simulink model "radia_ih"  (R2026a)
settings: Solver=FixedStepDiscrete  StopTime=1  FixedStep=0.10000000000000001
PreLoadFcn:
  | radia.simulink.makeIHMonitorBusObject();
InitFcn:
  | radia.simulink.updateIHGeometry(string(bdroot));
model workspace (MAT data in the model file):
  radia_ih_config.schema = 'radia.ih.simulink.native_sfunction.v1'
  radia_ih_config.backend = 'matlab-level2+radia-mex-handles'
  radia_ih_config.python_fallback = 0
  radia_ih_config.release_channel = "preview"
  radia_ih_config.operator_assembly = "diagnostic"
  radia_ih_config.diagnostic_only = 1
  radia_ih_config.eddy_solver = 'fem'
  radia_ih_config.thermal_solver = 'fem'
  radia_ih_config.n_eddy_unknown = 1
  radia_ih_config.n_heat = 1
  radia_ih_config.n_temperature = 1
  radia_ih_config.bh_mode = 'linear'
  radia_ih_config.eddy_matrix_real = 1
  radia_ih_config.eddy_matrix_imag = 0
  radia_ih_config.eddy_rhs_real = 1
  radia_ih_config.eddy_rhs_imag = 0
  radia_ih_config.heat_projection = 1
  radia_ih_config.heat_cell_weights = 1
  radia_ih_config.heat_to_temperature_projection = 1
  radia_ih_config.mass_row_ptr = [0; 1]
  radia_ih_config.mass_col = 0
  radia_ih_config.mass_value = 1
  radia_ih_config.stiffness_row_ptr = [0; 1]
  radia_ih_config.stiffness_col = 0
  radia_ih_config.stiffness_value = 0
  radia_ih_config.temperature_cell_weights = 1
  radia_ih_config.initial_temperature_K = 293.15
  radia_ih_config.sample_time_s = 0.1
  radia_ih_config.thermal_tolerance = 1e-12
  radia_ih_config.thermal_max_iterations = 100
  radia_ih_config.rotation_mode = 'periodic-uniform'
  radia_ih_config.angle_origin_rad = 0
  radia_ih_config.temperature_coordinate_system = "workpiece"
  radia_ih_config.rotation_transport = "conservative-periodic"
  radia_ih_config.dt_order = "eddy;transport(theta_prev,theta_now);thermal"
  radia_ih_config.convection_W_per_m2K = 0
  radia_ih_config.configured = 1
  radia_ih_config.distributed_field = 1
  radia_ih_config.surrogate = 0
  radia_ih_config.current_change_recomputes_eddy = 0
  radia_ih_config.temperature_change_recomputes_eddy = 0
  radia_ih_geometry_revision = nan
libraries: simulink x1
settings Model: Creator=Administrator  LastModifiedBy=Administrator

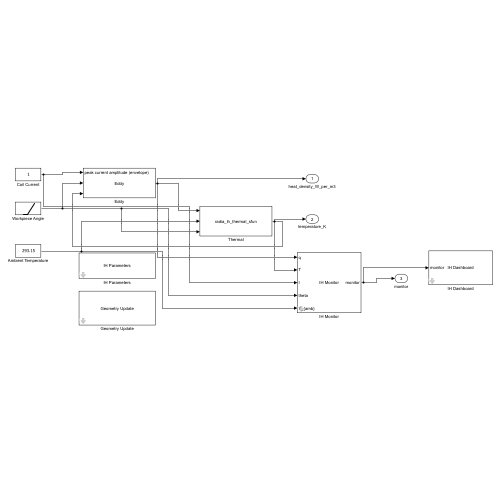
[thumbnail: Simulink's stored preview of the top-level diagram]
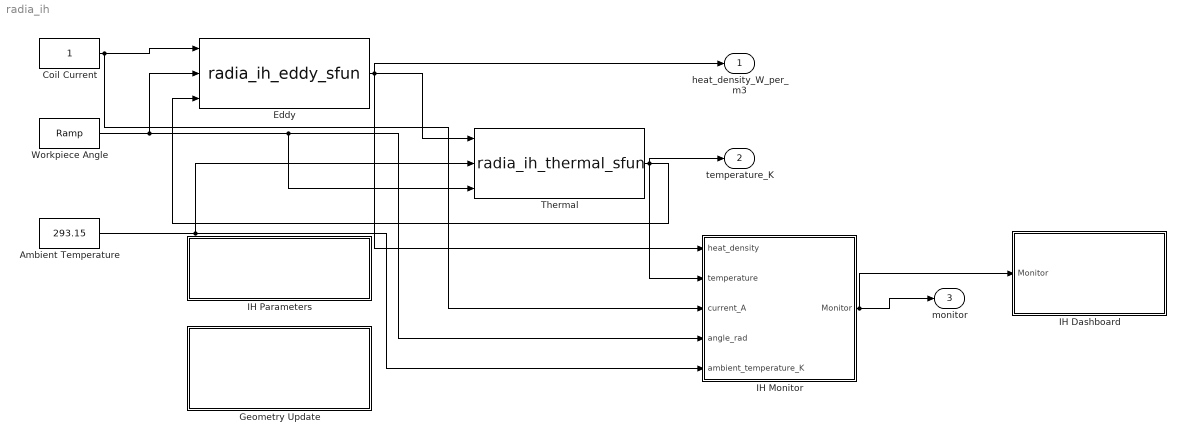
== system radia_ih ==
  Ambient Temperature : Constant  Value=293.15
  Coil Current : Constant
  Eddy : M-S-Function  FunctionName=radia_ih_eddy_sfun  Parameters=radia_ih_config
      mask help: Input 1 is peak current amplitude (envelope), not instantaneous carrier samples. Frozen per-panel ESIM rejects zero-start/soft-start ramps outside the reference band, which cannot be widened beyond 10%. Rebuild at another reference current.
      mask Display: disp('Eddy'); port_label('input',1,'peak current amplitude (envelope)');
  Geometry Update : Subsystem  Tag=RadiaIHGeometryUpdate  mask{wp_vol=, coil_file=, assemble_fcn=, assemble_command=, config_file=, frequency_hz=7000, coil_sigma=5.8e7, workpiece_sigma=5.0e6, workpiece_mu_r=100, density=7800, heat_capacity=467, thermal_conductivity=46.6, thermal_order=1, convection=10, initial_temperature_K=293.15, sample_time_s=0.5, workpiece_label=sibc, coil_body_label=body, coil_source_label=source, coil_sink_label=sink, peec_n_peri=16, coil_step_solver=peec, fin_n_lanes=, fin_n_stations=, fin_lane_grading=auto, fin_tip_lanes=, peec_proximity=on, coupling_mode=weak, workpiece_bem_backend=intree-dense, python_executable=python, axisymmetric_thermal_vol=, panel_zs_file=, n_phi_samples=128, auto_rebuild=on, zs_mode=uniform, esim_panel_evaluator=table, esim_bh_file=, esim_tolerance=1e-3, esim_max_iter=15, esim_half_thickness_m=0.01, esim_reference_phase_rad=0, esim_drive_relative_band=0.1, esim_reference_current_A=1}
      mask prompts: wp_vol "Workpiece mesh (.vol / .vol.gz)"; coil_file "Coil geometry (.step/.stp PEEC / .vol BEM-A)"; assemble_fcn "Custom assemble function (optional): fcn(wpVol, coilFile, configFile)"; assemble_command "Custom assemble command (optional; writes config_file)"; config_file "Configuration MAT/JSON (blank = derive from geometry)"; frequency_hz "Frequency (Hz)"; coil_sigma "Coil conductivity (S/m)"; workpiece_sigma "Workpiece conductivity (S/m)"; workpiece_mu_r "Workpiece relative permeability"; density "Density (kg/m^3)"; heat_capacity "Heat capacity (J/kg/K)"; thermal_conductivity "Thermal conductivity (W/m/K)"; thermal_order "Thermal H1 order"; convection "Convection coefficient (W/m^2/K)"; initial_temperature_K "Initial temperature (K)"; sample_time_s "Sample time (s)"; workpiece_label "Workpiece SIBC label (contract)"; coil_body_label "BEM-A body label (contract)"; coil_source_label "BEM-A source label (contract)"; coil_sink_label "BEM-A sink label (contract)"; peec_n_peri "PEEC perimeter filaments"; coil_step_solver "STEP coil solver"; fin_n_lanes "Fin surface lanes (blank: measured)"; fin_n_stations "Fin surface stations (blank: measured)"; fin_lane_grading "Fin lane grading"; fin_tip_lanes "Fin tip lanes (blank: measured)"; peec_proximity "PEEC proximity correction"; coupling_mode "Electromagnetic coupling"; workpiece_bem_backend "Workpiece BEM backend"; python_executable "Python executable (blank: radia.setup selection)"; axisymmetric_thermal_vol "Axisymmetric thermal .vol (blank: 3D heat)"; panel_zs_file "Element Zs JSON (ohm; blank: uniform SIBC)"; n_phi_samples "Azimuth samples for axisymmetric heat"; auto_rebuild "Rebuild automatically when files change"; zs_mode "Surface impedance mode"; esim_panel_evaluator "ESIM evaluator"; esim_bh_file "ESIM B-H input file"; esim_tolerance "ESIM outer relative tolerance"; esim_max_iter "ESIM outer iteration limit"; esim_half_thickness_m "ESIM half thickness (m)"; esim_reference_phase_rad "Frozen ESIM reference phase (rad; zero only)"; esim_drive_relative_band "Frozen ESIM allowed drive relative band (0 to 0.1)"; esim_reference_current_A "ESIM frozen reference current (A peak)"
      mask help: Watches geometry and assembly controls at explicit update/initialization. Per-panel ESIM freezes directly certified Zs at the declared peak reference current (phase zero) and frequency. Eddy input 1 is peak current amplitude (envelope), not carrier samples. Its allowed band cannot be widened beyond 10%; zero-start/soft-start outside that band raises. Rebuild at a new reference current. This is not nonlinear time stepping.
      mask TypeOptions thermal_order: 1 | 2
      mask TypeOptions coil_step_solver: peec | fin-surface
      mask TypeOptions fin_lane_grading: auto | uniform
      mask TypeOptions coupling_mode: weak | strong
      mask TypeOptions workpiece_bem_backend: intree-dense | hacapk
      mask TypeOptions zs_mode: uniform | element-file | per-panel-esim
      mask TypeOptions esim_panel_evaluator: table | direct
      mask DialogControl browse_wp_vol Prompt: Browse...
      mask DialogControl browse_wp_vol Tooltip: Select the workpiece Netgen .vol or .vol.gz mesh.
      mask DialogControl browse_wp_vol Callback: radia.simulink.browseIHGeometryFile(string(gcb), 'workpiece');
      mask DialogControl browse_coil_file Prompt: Browse...
      mask DialogControl browse_coil_file Tooltip: Select STEP CAD for PEEC or a .vol/.vol.gz mesh for BEM-A.
      mask DialogControl browse_coil_file Callback: radia.simulink.browseIHGeometryFile(string(gcb), 'coil');
      mask DialogControl rebuild_now Prompt: Rebuild now
      mask DialogControl rebuild_now Callback: radia.simulink.updateIHGeometry(string(bdroot(gcb)), Force=true);
      mask Display: disp('Geometry Update');
  IH Dashboard : Subsystem
      mask help: IH scalar telemetry dashboard. Distributed q and T remain separate physical outputs.
      mask Display: disp('IH Dashboard');port_label('input',1,'monitor');
  IH Monitor : Subsystem
      mask help: Native IH scalar telemetry. Internal signal reduction and Bus construction stay encapsulated; raw q and T remain separate.
      mask Display: disp('IH Monitor');port_label('input',1,'q');port_label('input',2,'T');port_label('input',3,'I');port_label('input',4,'theta');port_label('input',5,'T_{amb}');port_label('output',1,'monitor');
  IH Parameters : Subsystem  mask{config_file=}
      mask prompts: config_file "IH configuration MAT/JSON"
      mask help: Native IH preview configuration with preassembled operators. MAT files contain config or radia_ih_config; JSON is also supported.
      mask Callback config_file: radia.simulink.onIHConfigFileChanged(gcb);
      mask Display: disp('IH Parameters');
  Thermal : M-S-Function  FunctionName=radia_ih_thermal_sfun  Parameters=radia_ih_config
  Workpiece Angle : simulink/Sources/Ramp  slope=0  start=0  InitialOutput=0
  heat_density_W_per_m3 : Outport
  temperature_K : Outport  Port=2
  monitor : Outport  Port=3
  wires:
  Coil Current/1 -> Eddy/1, IH Monitor/3(current_A)
  Workpiece Angle/1 -> Thermal/3, IH Monitor/4(angle_rad), Eddy/2
  Ambient Temperature/1 -> Thermal/2, IH Monitor/5(ambient_temperature_K)
  Eddy/1 -> Thermal/1, heat_density_W_per_m3/1, IH Monitor/1(heat_density)
  Thermal/1 -> Eddy/3, temperature_K/1, IH Monitor/2(temperature)
  IH Monitor/1(Monitor) -> monitor/1, IH Dashboard/1(Monitor)

== system radia_ih/Geometry Update ==

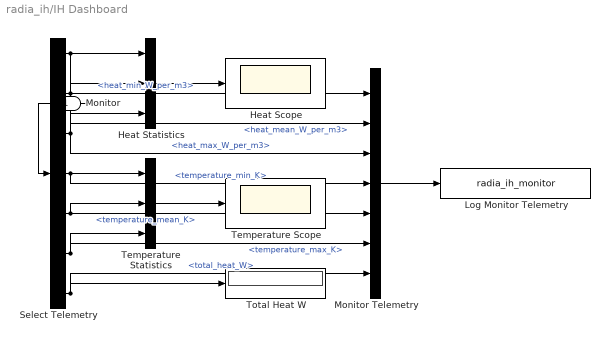
== system radia_ih/IH Dashboard ==
  Monitor : Inport
  Heat Scope : Scope
  Heat Statistics : Mux  Inputs=3
  Log Monitor Telemetry : ToWorkspace  VariableName=radia_ih_monitor  SampleTime=-1
  Monitor Telemetry : Mux  Inputs=7
  Select Telemetry : BusSelector  OutputSignals=heat_min_W_per_m3,heat_mean_W_per_m3,heat_max_W_per_m3,temperature_min_K,temperature_mean_K,temperature_max_K,total_heat_W
  Temperature Scope : Scope
  Temperature Statistics : Mux  Inputs=3
  Total Heat W : Display
  wires:
  Monitor/1 -> Select Telemetry/1
  Select Telemetry/1 -> Heat Statistics/1, Monitor Telemetry/1  "<heat_min_W_per_m3>"
  Select Telemetry/4 -> Temperature Statistics/1, Monitor Telemetry/4  "<temperature_min_K>"
  Select Telemetry/2 -> Heat Statistics/2, Monitor Telemetry/2  "<heat_mean_W_per_m3>"
  Select Telemetry/5 -> Temperature Statistics/2, Monitor Telemetry/5  "<temperature_mean_K>"
  Select Telemetry/3 -> Heat Statistics/3, Monitor Telemetry/3  "<heat_max_W_per_m3>"
  Select Telemetry/6 -> Temperature Statistics/3, Monitor Telemetry/6  "<temperature_max_K>"
  Select Telemetry/7 -> Monitor Telemetry/7, Total Heat W/1  "<total_heat_W>"
  Heat Statistics/1 -> Heat Scope/1
  Temperature Statistics/1 -> Temperature Scope/1
  Monitor Telemetry/1 -> Log Monitor Telemetry/1

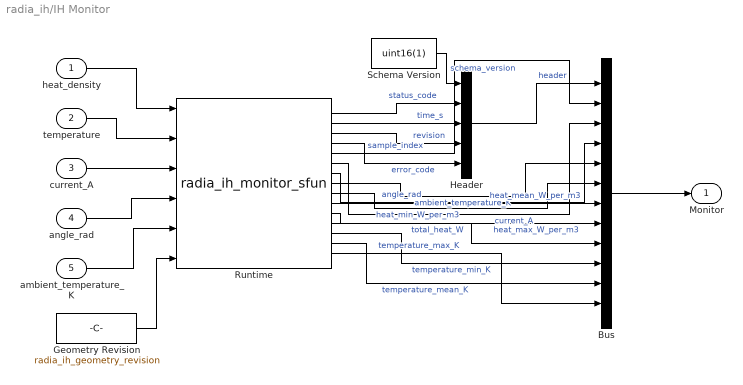
== system radia_ih/IH Monitor ==
  heat_density : Inport
  temperature : Inport  Port=2
  current_A : Inport  Port=3
  angle_rad : Inport  Port=4
  ambient_temperature_K : Inport  Port=5
  Bus : BusCreator  Inputs=12  OutDataTypeStr=Bus: IHMonitorBusV1  NonVirtualBus=on
  Geometry Revision : Constant  Value=radia_ih_geometry_revision
  Header : BusCreator  Inputs=5  OutDataTypeStr=Bus: RadiaMonitorHeaderV1  NonVirtualBus=on
  Runtime : M-S-Function  FunctionName=radia_ih_monitor_sfun  Parameters=radia_ih_config
  Schema Version : Constant  Value=uint16(1)  OutDataTypeStr=uint16
  Monitor : Outport
  wires:
  heat_density/1 -> Runtime/1
  temperature/1 -> Runtime/2
  current_A/1 -> Runtime/3
  angle_rad/1 -> Runtime/4
  ambient_temperature_K/1 -> Runtime/5
  Geometry Revision/1 -> Runtime/6
  Schema Version/1 -> Header/1  "schema_version"
  Runtime/1 -> Header/2  "status_code"
  Runtime/2 -> Header/3  "time_s"
  Runtime/3 -> Header/4  "revision"
  Runtime/4 -> Header/5  "error_code"
  Header/1 -> Bus/1  "header"
  Runtime/5 -> Bus/2  "sample_index"
  Runtime/6 -> Bus/3  "current_A"
  Runtime/7 -> Bus/4  "angle_rad"
  Runtime/8 -> Bus/5  "ambient_temperature_K"
  Runtime/9 -> Bus/6  "heat_min_W_per_m3"
  Runtime/10 -> Bus/7  "heat_mean_W_per_m3"
  Runtime/11 -> Bus/8  "heat_max_W_per_m3"
  Runtime/12 -> Bus/9  "total_heat_W"
  Runtime/13 -> Bus/10  "temperature_min_K"
  Runtime/14 -> Bus/11  "temperature_mean_K"
  Runtime/15 -> Bus/12  "temperature_max_K"
  Bus/1 -> Monitor/1

== system radia_ih/IH Parameters ==
